simulink model "ARDroneTTSim"  (R2017b)
settings: Solver=ode1  StartTime=0.0  StopTime=200  FixedStep=simDT  RelTol=1e-3  EnableMultiTasking=on
values from neighbouring files (symbols this model uses):
  timeDelay = FMS.Ts*4    [setupBaseModel.m]    (also in setupHoverSim.m; setupTTSim.m; setupWPTrackingSim.m)
undefined symbols (not defined in the file or in its folder): DiscIntNeverNeededParam, FMS, ssH, ssPitch, ssPitch2U, ssRoll, ssRoll2V, ssYaw
libraries: simulink x1, ARBlocks x1
settings Model: Creator=Paul Freeman  LastModifiedBy=ritac
settings DataIOCC: SaveFormat=Array  SignalLoggingSaveFormat=ModelDataLogs  SaveOutput=off  SignalLogging=off
settings OptimizationCC: ExpressionDepthLimit=2147483647  LifeSpan=inf
settings DebuggingCC: UnderspecifiedInitializationDetection=Classic  MergeDetectMultiDrivingBlocksExec=none  SolverPrmCheckMsg=warning  MultiTaskDSMMsg=warning  MultiTaskCondExecSysMsg=none  FcnCallInpInsideContextMsg=warning  AllowSymbolicDim=off  StateNameClashWarn=warning  SFUnexpectedBacktrackingDiag=warning  SFNoUnconditionalDefaultTransitionDiag=warning  SFExecutionAtInitializationDiag=none
settings HardwareCC: ProdBitPerPointer=32  ProdBitPerSizeT=32  ProdBitPerPtrDiffT=32  ProdLargestAtomicInteger=Long  ProdLargestAtomicFloat=Double  ProdEndianess=BigEndian  ProdWordSize=32  ProdHWDeviceType=Freescale->32-bit PowerPC
settings ModelReferenceCC: PropagateSignalLabelsOutOfModel=off
settings SFSimCC: SimParseCustomCode=off
settings CodeAppCC: StateflowObjectComments=on
settings GRTTargetCC: TargetLangStandard=C89/C90 (ANSI)  GeneratePreprocessorConditionals=Disable all  CombineOutputUpdateFcns=off  GRTInterface=on
settings ConfigComp: CovMetricSettings=dw  CovHtmlReporting=on  CovSaveCumulativeToWorkspaceVar=on  CovSaveSingleToWorkspaceVar=on  CovExternalEMLEnable=off

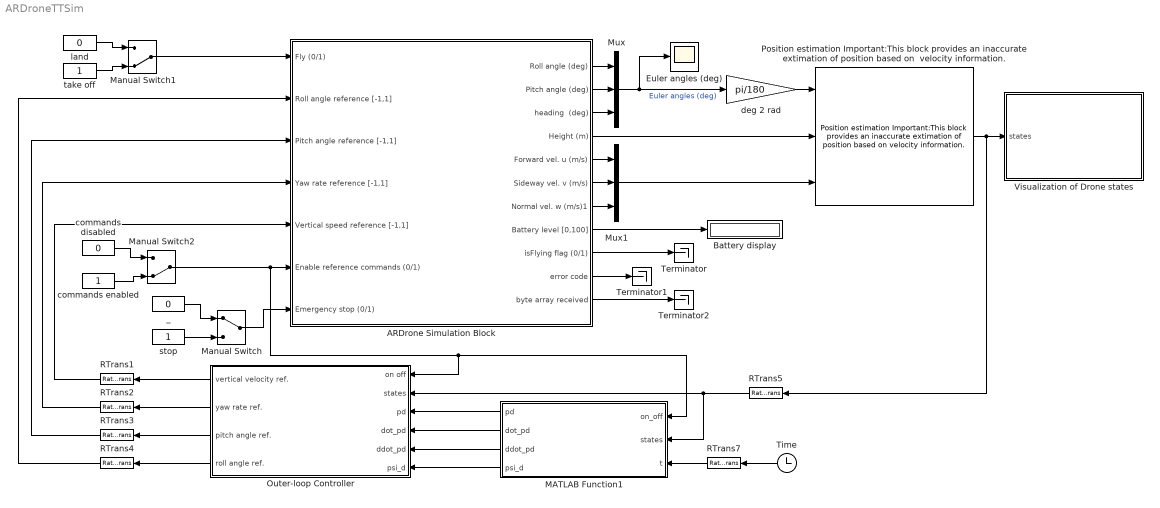
== system ARDroneTTSim ==
  ARDrone Simulation Block : Subsystem  AncestorBlock=ARBlocks/ARDrone Simulation Block
  Battery display : Display
  Euler angles (deg) : Scope
  MATLAB Function1 : MATLAB Function  TreatAsAtomicUnit=on  SystemSampleTime=FMS.Ts
  Manual Switch : ManualSwitch
  Manual Switch1 : ManualSwitch  CurrentSetting=0
  Manual Switch2 : ManualSwitch  CurrentSetting=0
  Mux : Mux  Inputs=3
  Mux1 : Mux  Inputs=3
  Outer-loop Controller : Subsystem
  "Position estimation Important:This block provides an inaccurate extimation of position based on  velocity information. " : ARBlocks/Position estimation Important:This block provides an  inaccurate extimation of position  based on  velocity information. 
  RTrans{1..4} (4 alike) : RateTransition  OutPortSampleTime=simDT
  RTrans5 : RateTransition  OutPortSampleTime=FMS.Ts
  RTrans7 : RateTransition  OutPortSampleTime=FMS.Ts
  Terminator : Terminator
  Terminator1 : Terminator
  Terminator2 : Terminator
  Time : Clock
  Visualization of Drone states : Subsystem
  _ : Constant  Value=0
  commands disabled : Constant  Value=0
  commands enabled : Constant
  deg 2 rad : Gain  Gain=pi/180
  land : Constant  Value=0
  stop : Constant
  take off : Constant
  wires:
  _/1 -> Manual Switch/1
  stop/1 -> Manual Switch/2
  land/1 -> Manual Switch1/1
  take off/1 -> Manual Switch1/2
  commands disabled/1 -> Manual Switch2/1
  commands enabled/1 -> Manual Switch2/2
  Manual Switch1/1 -> ARDrone Simulation Block/1(Fly (0/1))
  Manual Switch/1 -> ARDrone Simulation Block/7(Emergency stop (0/1))
  ARDrone Simulation Block/1(Roll angle (deg)) -> Mux/1
  ARDrone Simulation Block/2(Pitch angle (deg)) -> Mux/2
  ARDrone Simulation Block/5(Forward vel. u (m/s)) -> Mux1/1
  ARDrone Simulation Block/6(Sideway vel. v (m/s)) -> Mux1/2
  ARDrone Simulation Block/7(Normal vel. w (m/s)1) -> Mux1/3
  Mux/1 -> deg 2 rad/1, Euler angles (deg)/1  "Euler angles (deg)"
  ARDrone Simulation Block/8(Battery level [0,100]) -> Battery display/1
  "Position estimation Important:This block provides an inaccurate extimation of position based on  velocity information. "/1 -> RTrans5/1, Visualization of Drone states/1(states)
  deg 2 rad/1 -> "Position estimation Important:This block provides an inaccurate extimation of position based on  velocity information. "/1
  ARDrone Simulation Block/4(Height (m)) -> "Position estimation Important:This block provides an inaccurate extimation of position based on  velocity information. "/2
  Mux1/1 -> "Position estimation Important:This block provides an inaccurate extimation of position based on  velocity information. "/3
  Time/1 -> RTrans7/1
  ARDrone Simulation Block/3(heading  (deg)) -> Mux/3
  ARDrone Simulation Block/9(isFlying flag (0/1)) -> Terminator/1
  RTrans1/1 -> ARDrone Simulation Block/5(Vertical speed reference [-1,1])
  RTrans3/1 -> ARDrone Simulation Block/3(Pitch angle reference [-1,1])
  RTrans4/1 -> ARDrone Simulation Block/2(Roll angle reference [-1,1])
  RTrans7/1 -> MATLAB Function1/3(t)
  ARDrone Simulation Block/10(error code) -> Terminator1/1
  ARDrone Simulation Block/11(byte array received) -> Terminator2/1
  RTrans2/1 -> ARDrone Simulation Block/4(Yaw rate reference [-1,1])
  Manual Switch2/1 -> MATLAB Function1/1(on_off), Outer-loop Controller/1(on off), ARDrone Simulation Block/6(Enable reference commands (0/1))
  RTrans5/1 -> MATLAB Function1/2(states), Outer-loop Controller/2(states)
  MATLAB Function1/1(pd) -> Outer-loop Controller/3(pd)
  MATLAB Function1/2(dot_pd) -> Outer-loop Controller/4(dot_pd)
  MATLAB Function1/3(ddot_pd) -> Outer-loop Controller/5(ddot_pd)
  MATLAB Function1/4(psi_d) -> Outer-loop Controller/6(psi_d)
  Outer-loop Controller/1(vertical velocity ref.) -> RTrans1/1
  Outer-loop Controller/2(yaw rate ref.) -> RTrans2/1
  Outer-loop Controller/3(pitch angle ref.) -> RTrans3/1
  Outer-loop Controller/4(roll angle ref.) -> RTrans4/1

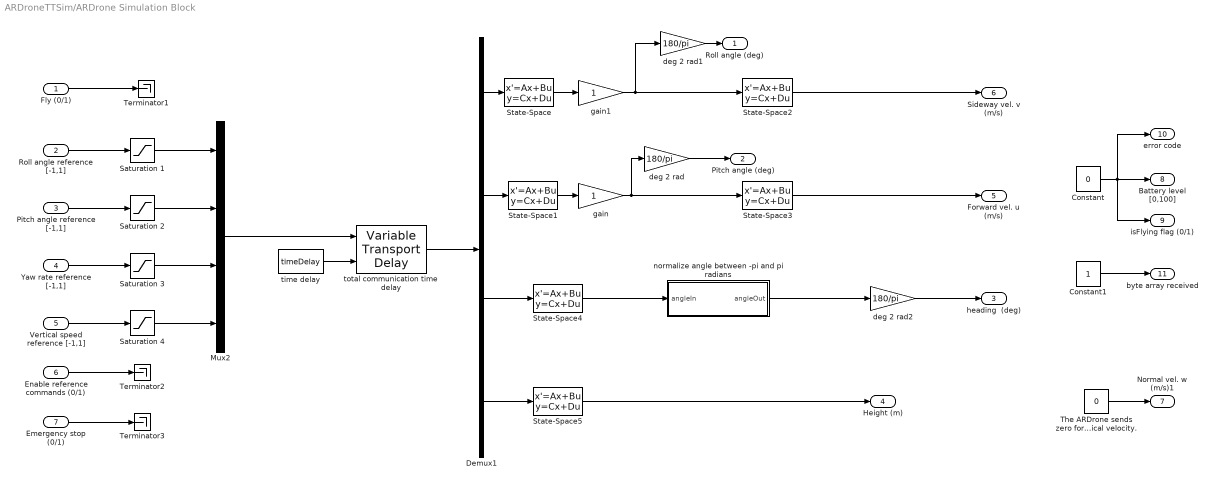
== system ARDroneTTSim/ARDrone Simulation Block ==
  Fly (0/1) : Inport
  Roll angle reference [-1,1] : Inport  Port=2
  Pitch angle reference [-1,1] : Inport  Port=3
  Yaw rate reference [-1,1] : Inport  Port=4
  Vertical speed reference [-1,1] : Inport  Port=5
  Enable reference commands (0/1) : Inport  Port=6
  Emergency stop (0/1) : Inport  Port=7
  Constant : Constant  Value=0
  Constant1 : Constant
  Demux1 : Demux  Outputs=[1,1,1,1]
  Mux2 : Mux  Inputs=[1,1,1,1]
  Saturation {1..4} (4 alike) : Saturate  UpperLimit=1  LowerLimit=-1
  State-Space : StateSpace  A=ssRoll.a  B=ssRoll.b  C=ssRoll.c  D=ssRoll.d  InitialCondition=0
  State-Space1 : StateSpace  A=ssPitch.a  B=ssPitch.b  C=ssPitch.c  D=ssPitch.d  InitialCondition=0
  State-Space2 : StateSpace  A=ssRoll2V.a  B=ssRoll2V.b  C=ssRoll2V.c  D=ssRoll2V.d  InitialCondition=0
  State-Space3 : StateSpace  A=ssPitch2U.a  B=ssPitch2U.b  C=ssPitch2U.c  D=ssPitch2U.d  InitialCondition=0
  State-Space4 : StateSpace  A=ssYaw.a  B=ssYaw.b  C=ssYaw.c  D=ssYaw.d  InitialCondition=0
  State-Space5 : StateSpace  A=ssH.a  B=ssH.b  C=ssH.c  D=ssH.d  InitialCondition=0
  Terminator1 : Terminator
  Terminator2 : Terminator
  Terminator3 : Terminator
  "The ARDrone sends zero for the vertical velocity. " : Constant  Value=0
  deg 2 rad : Gain  Gain=180/pi
  deg 2 rad1 : Gain  Gain=180/pi
  deg 2 rad2 : Gain  Gain=180/pi
  gain : Gain
  gain1 : Gain
  normalize angle between -pi and pi radians : MATLAB Function  TreatAsAtomicUnit=on
  time delay : Constant  Value=timeDelay
  total communication time delay : VariableTransportDelay  MaximumDelay=10  InitialOutput=[0 0 0 0]  MaximumPoints=4096
  Roll angle (deg) : Outport
  Pitch angle (deg) : Outport  Port=2
  heading  (deg) : Outport  Port=3
  Height (m) : Outport  Port=4
  Forward vel. u (m/s) : Outport  Port=5
  Sideway vel. v (m/s) : Outport  Port=6
  Normal vel. w (m/s)1 : Outport  Port=7
  Battery level [0,100] : Outport  Port=8
  isFlying flag (0/1) : Outport  Port=9
  error code : Outport  Port=10
  byte array received : Outport  Port=11
  wires:
  "The ARDrone sends zero for the vertical velocity. "/1 -> Normal vel. w (m/s)1/1
  Constant1/1 -> byte array received/1
  deg 2 rad2/1 -> heading  (deg)/1
  deg 2 rad1/1 -> Roll angle (deg)/1
  deg 2 rad/1 -> Pitch angle (deg)/1
  Constant/1 -> Battery level [0,100]/1, error code/1, isFlying flag (0/1)/1
  State-Space4/1 -> normalize angle between -pi and pi radians/1(angleIn)
  State-Space5/1 -> Height (m)/1
  Emergency stop (0/1)/1 -> Terminator3/1
  Enable reference commands (0/1)/1 -> Terminator2/1
  Fly (0/1)/1 -> Terminator1/1
  Demux1/3 -> State-Space4/1
  Demux1/2 -> State-Space1/1
  Saturation 4/1 -> Mux2/4
  Saturation 3/1 -> Mux2/3
  Saturation 2/1 -> Mux2/2
  Saturation 1/1 -> Mux2/1
  total communication time delay/1 -> Demux1/1
  Mux2/1 -> total communication time delay/1
  time delay/1 -> total communication time delay/2
  State-Space1/1 -> gain/1
  State-Space/1 -> gain1/1
  Demux1/4 -> State-Space5/1
  Demux1/1 -> State-Space/1
  Vertical speed reference [-1,1]/1 -> Saturation 4/1
  Yaw rate reference [-1,1]/1 -> Saturation 3/1
  Pitch angle reference [-1,1]/1 -> Saturation 2/1
  Roll angle reference [-1,1]/1 -> Saturation 1/1
  gain/1 -> State-Space3/1, deg 2 rad/1
  gain1/1 -> State-Space2/1, deg 2 rad1/1
  State-Space2/1 -> Sideway vel. v (m/s)/1
  State-Space3/1 -> Forward vel. u (m/s)/1
  normalize angle between -pi and pi radians/1(angleOut) -> deg 2 rad2/1

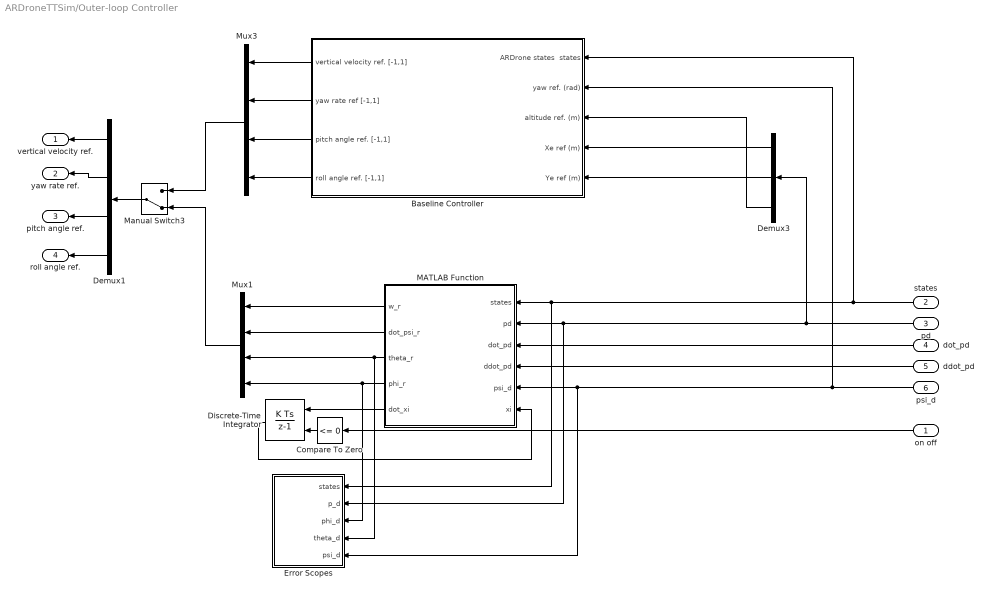
== system ARDroneTTSim/Outer-loop Controller ==
  on off : Inport  PortDimensions=1
  states : Inport  Port=2
  pd : Inport  Port=3  PortDimensions=[3 1]
  dot_pd : Inport  Port=4  PortDimensions=[3 1]
  ddot_pd : Inport  Port=5  PortDimensions=[3 1]
  psi_d : Inport  Port=6  PortDimensions=1
  Baseline Controller : Subsystem  AncestorBlock=ARBlocks/Baseline Controller
  Compare To Zero : simulink/Logic and Bit Operations/Compare To Zero  relop=<=  OutDataTypeStr=boolean
  Demux1 : Demux  Outputs=[1,1,1,1]
  Demux3 : Demux  Outputs=[1,1,1]
  Discrete-Time Integrator : DiscreteIntegrator  ExternalReset=level  InitialCondition=[0;0;0;0]  InitialConditionSetting=State (most efficient)  SampleTime=FMS.Ts  UpperSaturationLimit=10  LowerSaturationLimit=-10  ICPrevOutput=DiscIntNeverNeededParam  ICPrevScaledInput=DiscIntNeverNeededParam
  Error Scopes : Subsystem
  MATLAB Function : MATLAB Function  TreatAsAtomicUnit=on  SystemSampleTime=FMS.Ts
  Manual Switch3 : ManualSwitch  CurrentSetting=0
  Mux1 : Mux  Inputs=[1,1,1,1]
  Mux3 : Mux  Inputs=[1,1,1,1]
  vertical velocity ref. : Outport
  yaw rate ref. : Outport  Port=2
  pitch angle ref. : Outport  Port=3
  roll angle ref. : Outport  Port=4
  wires:
  states/1 -> Baseline Controller/1("ARDrone states  states "), Error Scopes/1(states), MATLAB Function/1(states)
  MATLAB Function/1(w_r) -> Mux1/1
  MATLAB Function/3(theta_r) -> Mux1/3, Error Scopes/4(theta_d)
  MATLAB Function/4(phi_r) -> Mux1/4, Error Scopes/3(phi_d)
  MATLAB Function/2(dot_psi_r) -> Mux1/2
  MATLAB Function/5(dot_xi) -> Discrete-Time Integrator/1
  Discrete-Time Integrator/1 -> MATLAB Function/6(xi)
  pd/1 -> Demux3/1, Error Scopes/2(p_d), MATLAB Function/2(pd)
  dot_pd/1 -> MATLAB Function/3(dot_pd)
  ddot_pd/1 -> MATLAB Function/4(ddot_pd)
  psi_d/1 -> Error Scopes/5(psi_d), MATLAB Function/5(psi_d), Baseline Controller/2(yaw ref. (rad))
  Demux3/1 -> Baseline Controller/4(Xe ref (m))
  Demux3/2 -> Baseline Controller/5(Ye ref (m))
  Demux3/3 -> Baseline Controller/3(altitude ref. (m))
  Baseline Controller/4(roll angle ref. [-1,1]) -> Mux3/4
  Baseline Controller/3(pitch angle ref. [-1,1]) -> Mux3/3
  Baseline Controller/2(yaw rate ref [-1,1]) -> Mux3/2
  Baseline Controller/1(vertical velocity ref. [-1,1]) -> Mux3/1
  Mux3/1 -> Manual Switch3/1
  Demux1/1 -> vertical velocity ref./1
  Demux1/2 -> yaw rate ref./1
  Demux1/3 -> pitch angle ref./1
  Demux1/4 -> roll angle ref./1
  Manual Switch3/1 -> Demux1/1
  Mux1/1 -> Manual Switch3/2
  on off/1 -> Compare To Zero/1
  Compare To Zero/1 -> Discrete-Time Integrator/2

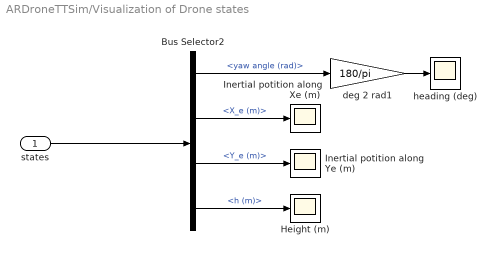
== system ARDroneTTSim/Visualization of Drone states ==
  states : Inport
  Bus Selector2 : BusSelector  OutputSignals=yaw angle (rad),X_e (m),Y_e (m),h (m)
  Height (m) : Scope
  Inertial potition along Xe (m) : Scope
  Inertial potition along Ye (m) : Scope
  deg 2 rad1 : Gain  Gain=180/pi
  heading (deg) : Scope
  wires:
  states/1 -> Bus Selector2/1
  Bus Selector2/1 -> deg 2 rad1/1  "<yaw angle (rad)>"
  Bus Selector2/2 -> Inertial potition along Xe (m)/1  "<X_e (m)>"
  Bus Selector2/3 -> Inertial potition along Ye (m)/1  "<Y_e (m)>"
  Bus Selector2/4 -> Height (m)/1  "<h (m)>"
  deg 2 rad1/1 -> heading (deg)/1

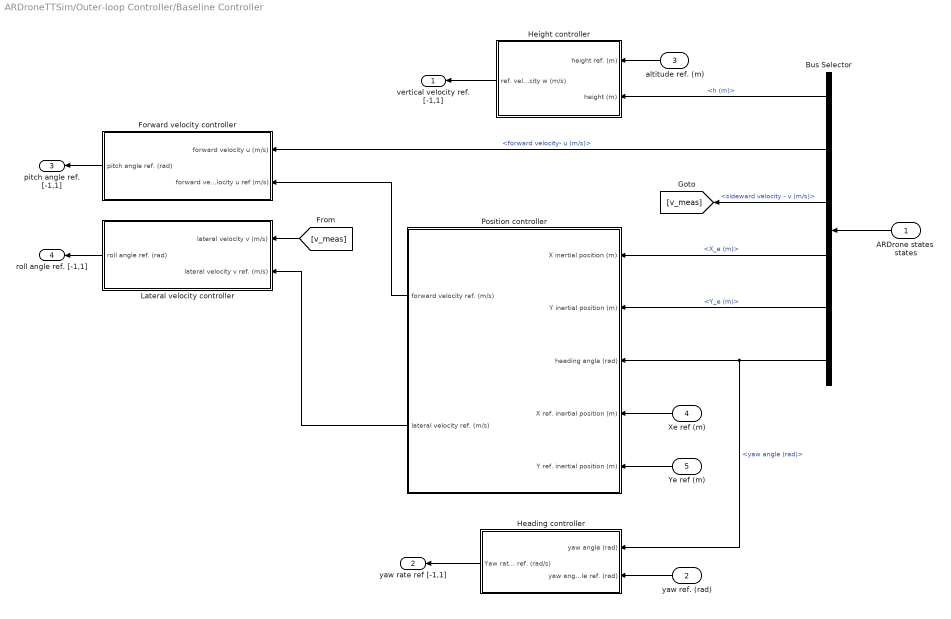
== system ARDroneTTSim/Outer-loop Controller/Baseline Controller ==
  "ARDrone states  states " : Inport
  yaw ref. (rad) : Inport  Port=2
  altitude ref. (m) : Inport  Port=3
  Xe ref (m) : Inport  Port=4
  Ye ref (m) : Inport  Port=5
  Bus Selector : BusSelector  OutputSignals=h (m),forward velocity- u (m/s),sideward velocity - v (m/s),X_e (m),Y_e (m),yaw angle (rad)
  "Forward velocity controller " : Subsystem
  Heading controller : Subsystem
  "Height controller " : Subsystem
  Lateral velocity controller : Subsystem
  Position controller : Subsystem
  vertical velocity ref. [-1,1] : Outport
  yaw rate ref [-1,1] : Outport  Port=2
  pitch angle ref. [-1,1] : Outport  Port=3
  roll angle ref. [-1,1] : Outport  Port=4
  wires:
  [v_meas] -> Lateral velocity controller/1(lateral velocity v (m/s))
  Bus Selector/3 -> [v_meas]  "<sideward velocity - v (m/s)>"
  Position controller/2(lateral velocity ref. (m/s)) -> Lateral velocity controller/2(lateral velocity v ref. (m/s))
  Position controller/1(forward velocity ref. (m/s)) -> "Forward velocity controller "/2(forward velocity u ref (m/s))
  Ye ref (m)/1 -> Position controller/5(Y ref. inertial position (m))
  Xe ref (m)/1 -> Position controller/4(X ref. inertial position (m))
  Bus Selector/5 -> Position controller/2(Y inertial position (m))  "<Y_e (m)>"
  Bus Selector/4 -> Position controller/1(X inertial position (m))  "<X_e (m)>"
  Heading controller/1(Yaw rate ref. (rad/s)) -> yaw rate ref [-1,1]/1
  yaw ref. (rad)/1 -> Heading controller/2(yaw angle ref. (rad))
  "Forward velocity controller "/1(pitch angle ref. (rad)) -> pitch angle ref. [-1,1]/1
  Bus Selector/2 -> "Forward velocity controller "/1(forward velocity u (m/s))  "<forward velocity- u (m/s)>"
  Lateral velocity controller/1(roll angle ref. (rad)) -> roll angle ref. [-1,1]/1
  "Height controller "/1(ref. velocity w (m/s)) -> vertical velocity ref. [-1,1]/1
  Bus Selector/1 -> "Height controller "/2(height (m))  "<h (m)>"
  altitude ref. (m)/1 -> "Height controller "/1(height ref. (m))
  "ARDrone states  states "/1 -> Bus Selector/1
  Bus Selector/6 -> Position controller/3(heading angle (rad)), Heading controller/1(yaw angle (rad))  "<yaw angle (rad)>"

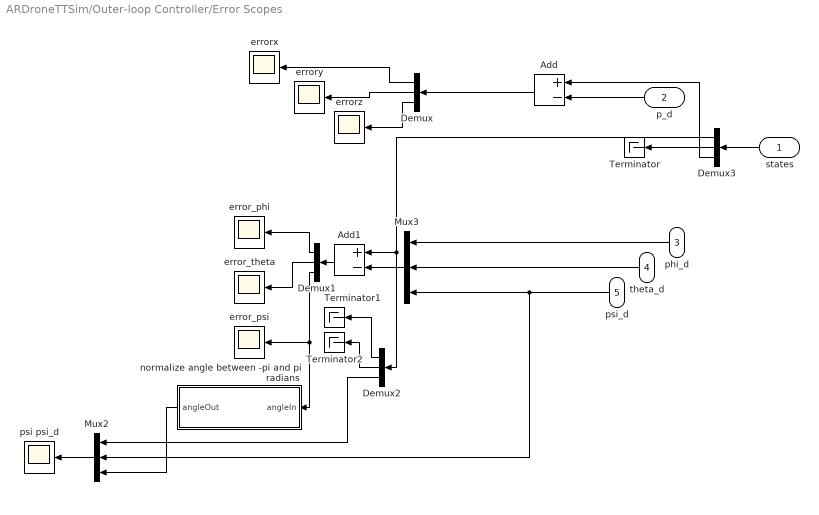
== system ARDroneTTSim/Outer-loop Controller/Error Scopes ==
  states : Inport
  p_d : Inport  Port=2
  phi_d : Inport  Port=3
  theta_d : Inport  Port=4
  psi_d : Inport  Port=5
  Add : Sum  Inputs=+-
  Add1 : Sum  Inputs=+-
  Demux : Demux  Outputs=3
  Demux1 : Demux  Outputs=[1,1,1]
  Demux2 : Demux  Outputs=[1,1,1]
  Demux3 : Demux  Outputs=[3,3,3]
  Mux2 : Mux  Inputs=[1,1,1]
  Mux3 : Mux  Inputs=[1,1,1]
  Terminator : Terminator
  Terminator1 : Terminator
  Terminator2 : Terminator
  error_phi : Scope
  error_psi : Scope
  error_theta : Scope
  errorx : Scope
  errory : Scope
  errorz : Scope
  normalize angle between -pi and pi radians : MATLAB Function  TreatAsAtomicUnit=on
  psi psi_d : Scope
  wires:
  Add/1 -> Demux/1
  Demux/1 -> errorx/1
  Demux/3 -> errorz/1
  Demux/2 -> errory/1
  Demux1/1 -> error_phi/1
  Demux1/2 -> error_theta/1
  p_d/1 -> Add/2
  phi_d/1 -> Mux3/1
  theta_d/1 -> Mux3/2
  psi_d/1 -> Mux2/2, Mux3/3
  Mux2/1 -> psi psi_d/1
  Demux1/3 -> normalize angle between -pi and pi radians/1(angleIn), error_psi/1
  Demux2/3 -> Mux2/1
  normalize angle between -pi and pi radians/1(angleOut) -> Mux2/3
  states/1 -> Demux3/1
  Demux3/3 -> Add/1
  Demux3/1 -> Add1/1, Demux2/1
  Add1/1 -> Demux1/1
  Mux3/1 -> Add1/2
  Demux3/2 -> Terminator/1
  Demux2/1 -> Terminator1/1
  Demux2/2 -> Terminator2/1

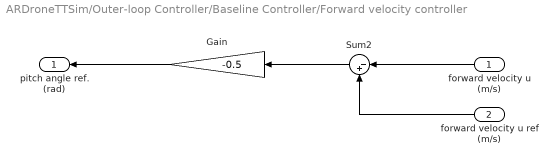
== system ARDroneTTSim/Outer-loop Controller/Baseline Controller/Forward velocity controller  ==
  forward velocity u (m/s) : Inport
  forward velocity u ref (m/s) : Inport  Port=2
  Gain : Gain  Gain=-0.5
  Sum2 : Sum  Inputs=|-+
  pitch angle ref. (rad) : Outport
  wires:
  forward velocity u ref (m/s)/1 -> Sum2/2
  Gain/1 -> pitch angle ref. (rad)/1
  Sum2/1 -> Gain/1
  forward velocity u (m/s)/1 -> Sum2/1

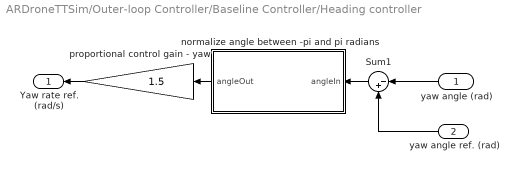
== system ARDroneTTSim/Outer-loop Controller/Baseline Controller/Heading controller ==
  yaw angle (rad) : Inport
  yaw angle ref. (rad) : Inport  Port=2
  Sum1 : Sum  Inputs=|-+
  normalize angle between -pi and pi radians : MATLAB Function  TreatAsAtomicUnit=on
  proportional control gain - yaw : Gain  Gain=1.5
  Yaw rate ref. (rad/s) : Outport
  wires:
  yaw angle ref. (rad)/1 -> Sum1/2
  proportional control gain - yaw/1 -> Yaw rate ref. (rad/s)/1
  yaw angle (rad)/1 -> Sum1/1
  normalize angle between -pi and pi radians/1(angleOut) -> proportional control gain - yaw/1
  Sum1/1 -> normalize angle between -pi and pi radians/1(angleIn)

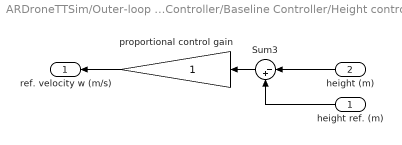
== system ARDroneTTSim/Outer-loop Controller/Baseline Controller/Height controller  ==
  height ref. (m) : Inport
  height (m) : Inport  Port=2
  Sum3 : Sum  Inputs=|-+
  proportional control gain : Gain
  ref. velocity w (m/s) : Outport
  wires:
  height ref. (m)/1 -> Sum3/2
  height (m)/1 -> Sum3/1
  Sum3/1 -> proportional control gain/1
  proportional control gain/1 -> ref. velocity w (m/s)/1

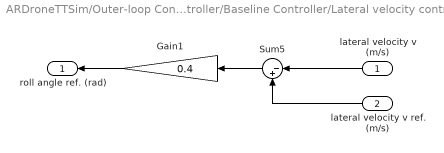
== system ARDroneTTSim/Outer-loop Controller/Baseline Controller/Lateral velocity controller ==
  lateral velocity v (m/s) : Inport
  lateral velocity v ref. (m/s) : Inport  Port=2
  Gain1 : Gain  Gain=0.4
  Sum5 : Sum  Inputs=|-+
  roll angle ref. (rad) : Outport
  wires:
  lateral velocity v ref. (m/s)/1 -> Sum5/2
  Gain1/1 -> roll angle ref. (rad)/1
  Sum5/1 -> Gain1/1
  lateral velocity v (m/s)/1 -> Sum5/1

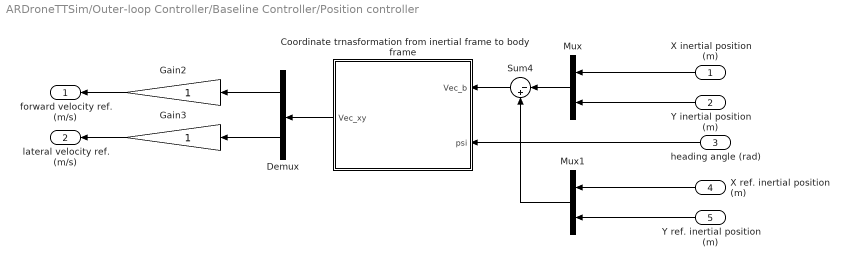
== system ARDroneTTSim/Outer-loop Controller/Baseline Controller/Position controller ==
  X inertial position (m) : Inport
  Y inertial position (m) : Inport  Port=2
  heading angle (rad) : Inport  Port=3
  X ref. inertial position (m) : Inport  Port=4
  Y ref. inertial position (m) : Inport  Port=5
  "Coordinate trnasformation from inertial frame to body frame " : MATLAB Function  TreatAsAtomicUnit=on
  Demux : Demux  Outputs=2
  Gain2 : Gain
  Gain3 : Gain
  Mux : Mux  Inputs=2
  Mux1 : Mux  Inputs=2
  Sum4 : Sum  Inputs=|-+
  forward velocity ref. (m/s) : Outport
  lateral velocity ref. (m/s) : Outport  Port=2
  wires:
  Gain3/1 -> lateral velocity ref. (m/s)/1
  Demux/2 -> Gain3/1
  Demux/1 -> Gain2/1
  Y ref. inertial position (m)/1 -> Mux1/2
  X ref. inertial position (m)/1 -> Mux1/1
  Mux/1 -> Sum4/1
  X inertial position (m)/1 -> Mux/1
  Y inertial position (m)/1 -> Mux/2
  Sum4/1 -> "Coordinate trnasformation from inertial frame to body frame "/1(Vec_b)
  Mux1/1 -> Sum4/2
  "Coordinate trnasformation from inertial frame to body frame "/1(Vec_xy) -> Demux/1
  heading angle (rad)/1 -> "Coordinate trnasformation from inertial frame to body frame "/2(psi)
  Gain2/1 -> forward velocity ref. (m/s)/1

== matlab function ARDroneTTSim/MATLAB Function1 ==
  data: on_off input; states input; t input; pd output; dot_pd output; ddot_pd output; psi_d output
function [pd, dot_pd, ddot_pd, psi_d] = desired_trajectory(on_off,states,t)
%#codegen

% ------------------------------------------------------------------------
% inputs:
% on_off - 1 if tracking is on, 0 if it is off
% states - structure with state variables
% t - current simulation time
% 
% outputs:
% pd - desired position
% dot_pd - desired velocity
% ddot_pd - desired acceleration
% psi_d - desired yaw angle
% ------------------------------------------------------------------------

persistent t0
persistent p0
persistent previous_status

on = 1;
off = 0;

if isempty(previous_status)
    previous_status = on;
    p0 = [states(7:8);-1];
end

if on_off == off
    if previous_status == on 
    % first time off or switching back off
        p0 = [states(7:8);-1]; % x0 and y0 match the current position
    end
    pd = p0;
    dot_pd = [0;0;0];
    ddot_pd = [0;0;0];
    psi_d = 0;
else
    if isempty(t0) || (previous_status == off) 
    % first time on or switching back on
        t0 = t;
        p0 = [states(7:8);-1];
    end
    dt = t-t0;

%!!!!!!!!!!!!!!!!!!!!!!!!!!!!!!!!!!!!!!!!!!!!!!!!!!!!!!!!!!!!!!!!!!!!!!!!
% replace with the necessary code to define adequate desired trajectories
% use dt, p0, and any additional parameters
    pd = p0;
    dot_pd = [0;0;0];
    ddot_pd = [0;0;0];
    psi_d = 0;
%!!!!!!!!!!!!!!!!!!!!!!!!!!!!!!!!!!!!!!!!!!!!!!!!!!!!!!!!!!!!!!!!!!!!!!!!

end

previous_status = on_off;

== matlab function ARDroneTTSim/Outer-loop Controller/MATLAB Function ==
  data: w_r output; dot_psi_r output; theta_r output; states input; pd input; dot_pd input; ddot_pd input; psi_d input; xi input; phi_r output; dot_xi output
function [w_r, dot_psi_r, theta_r, phi_r, dot_xi] = tt_controller(states, pd, dot_pd, ddot_pd,psi_d,xi)
%#codegen

% ------------------------------------------------------------------------
% inputs:
% states - structure with state variables
% pd - desired position
% dot_pd - desired velocity
% ddot_pt - desired acceleration
% psi_d - desired yaw angle
% xi - integral state (four variables)
%
% outputs:
% w_r - vertical velocity reference
% dot_psi_r - yaw rate reference
% theta_r - pitch angle reference
% phi_r - roll angle reference
% dot_xi - integral state derivative
% ------------------------------------------------------------------------

lambda = states(1:3,1); % Euler angles
psi = lambda(3);
R=euler2R(lambda);
Rz = [cos(psi) -sin(psi) 0; sin(psi) cos(psi) 0; 0 0 1];
psi_e = normalize_angle(psi-psi_d);

p = states(7:9,1); % position vector
p(3) = -p(3); % height is symmetric of z
vb = states(4:6,1); % velocity vector in body coordinates
dot_p = R*vb; % body velocity rotated to inertial frame 
dot_p(3) = -dot_p(3);

%!!!!!!!!!!!!!!!!!!!!!!!!!!!!!!!!!!!!!!!!!!!!!!!!!!!!!!!!!!!!!!!!!!!!!!
% replace with the necessary code to implement the trajectory tracking
% controller
w_r= 0;
dot_psi_r = 0;
theta_r = 0;
phi_r = 0;
dot_xi = [0;0;0;0];
%!!!!!!!!!!!!!!!!!!!!!!!!!!!!!!!!!!!!!!!!!!!!!!!!!!!!!!!!!!!!!!!!!!!!!!


function R = euler2R(l)
%#codegen
% returns the rotation matrix for a given vector of euler angles

phi = l(1); theta = l(2); psi = l(3);
R = [cos(theta)*cos(psi)...
      sin(phi)*sin(theta)*cos(psi)-cos(phi)*sin(psi)...
      cos(phi)*sin(theta)*cos(psi)+sin(phi)*sin(psi);
   cos(theta)*sin(psi)...
   sin(phi)*sin(theta)*sin(psi)+cos(phi)*cos(psi)... 
   cos(phi)*sin(theta)*sin(psi)-sin(phi)*cos(psi);
   -sin(theta)...
   sin(phi)*cos(theta)...
   cos(phi)*cos(theta)];

function angleOut = normalize_angle(angleIn)
%#codegen

angleOut = mod(angleIn, 2*pi) ;
if angleOut > pi
    angleOut = -2*pi + angleOut ; 
end

== matlab function ARDroneTTSim/Outer-loop Controller/Baseline Controller/Heading controller/normalize angle between -pi and pi radians ==
  data: angleIn input; angleOut output
function angleOut = fcn(angleIn)
%#codegen

angleOut = mod(angleIn, 2*pi) ;
if angleOut > pi
    angleOut = -2*pi + angleOut ; 
end

== matlab function ARDroneTTSim/ARDrone Simulation Block/normalize angle between -pi and pi radians ==
  data: angleIn input; angleOut output
function angleOut = fcn(angleIn)
%#codegen

angleOut = mod(angleIn, 2*pi) ;
if angleOut > pi
    angleOut = -2*pi + angleOut ; 
end

== matlab function ARDroneTTSim/Outer-loop Controller/Error Scopes/normalize angle between -pi and pi radians ==
  data: angleIn input; angleOut output
function angleOut = fcn(angleIn)
%#codegen

angleOut = mod(angleIn, 2*pi) ;
if angleOut > pi
    angleOut = -2*pi + angleOut ; 
end

== matlab function ARDroneTTSim/Outer-loop Controller/Baseline Controller/Position controller/Coordinate trnasformation from inertial frame to body frame  ==
  data: Vec_b input; Vec_xy output; psi input
function Vec_xy  = fcn(Vec_b , psi)
%#codegen
T = [cos(psi) sin(psi) ; -sin(psi) cos(psi)] ; 
Vec_xy = T*Vec_b(1:2,1);
